simulink model "temp_sensor"  (R2025b)
settings: Solver=VariableStepAuto  StartTime=0.0  StopTime=10.0  RelTol=1e-3
undefined symbols (not defined in the file): dspblkCoreblockFVToolHelper, gcbh
libraries: arduinolib x2
settings Model: Creator=00782620  LastModifiedBy=00782620

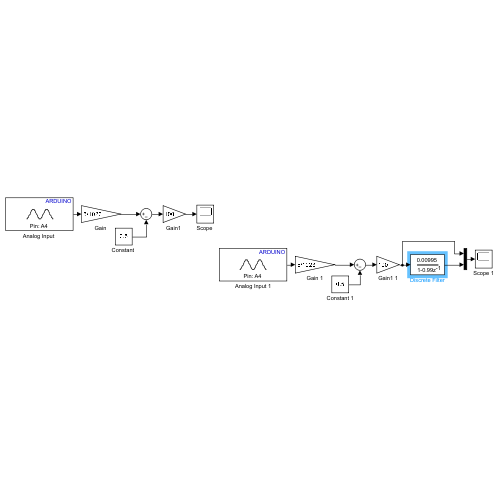
[thumbnail: Simulink's stored preview of the top-level diagram]
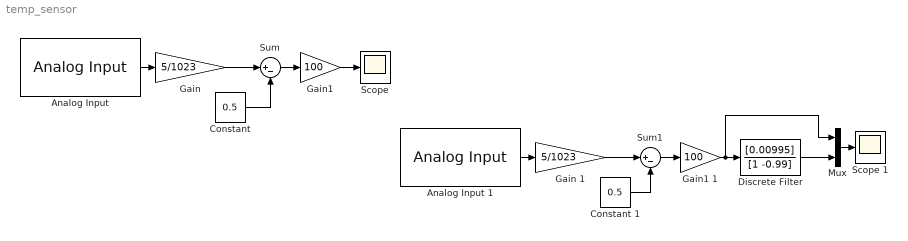
== system temp_sensor ==
  "Analog Input " : arduinolib/Analog Input  pinNumber=4  ReadResultsOnly=off  ConversionTriggerSource=Software  ExternalTriggerType=uint32( 0 )  OutputDataType=uint16  EnableConversionCompleteNotify=off  EnableOuputStatus=off  SampleTime=0.01  blockPlatform=arduino
  Analog Input 1 : arduinolib/Analog Input  pinNumber=4  ReadResultsOnly=off  ConversionTriggerSource=Software  ExternalTriggerType=uint32( 0 )  OutputDataType=uint16  EnableConversionCompleteNotify=off  EnableOuputStatus=off  SampleTime=0.01  blockPlatform=arduino
  "Constant " : Constant  Value=0.5
  Constant 1 : Constant  Value=0.5
  Discrete Filter : DiscreteFilter  LoadFcn=dspblkCoreblockFVToolHelper(gcbh,'load');  Numerator=[0.00995]  Denominator=[1 -0.99]
      settings: CopyFcn=dspblkCoreblockFVToolHelper(gcbh,'copy');  DeleteFcn=dspblkCoreblockFVToolHelper(gcbh,'close');  ModelCloseFcn=dspblkCoreblockFVToolHelper(gcbh,'close');  PreSaveFcn=dspblkCoreblockFVToolHelper(gcbh,'presave');  PostSaveFcn=dspblkCoreblockFVToolHelper(gcbh,'postsave');  CloseFcn=dspblkCoreblockFVToolHelper(gcbh,'close');
  "Gain " : Gain  Gain=5/1023
  Gain 1 : Gain  Gain=5/1023
  "Gain1 " : Gain  Gain=100
  Gain1 1 : Gain  Gain=100
  Mux : Mux  Inputs=2
  "Scope " : Scope
  Scope 1 : Scope
  Sum : Sum  Inputs=|+-
  Sum1 : Sum  Inputs=|+-
  wires:
  "Analog Input "/1 -> "Gain "/1
  "Gain "/1 -> Sum/1
  "Constant "/1 -> Sum/2
  Sum/1 -> "Gain1 "/1
  "Gain1 "/1 -> "Scope "/1
  Sum1/1 -> Gain1 1/1
  Constant 1/1 -> Sum1/2
  Gain 1/1 -> Sum1/1
  Analog Input 1/1 -> Gain 1/1
  Gain1 1/1 -> Mux/1, Discrete Filter/1
  Discrete Filter/1 -> Mux/2
  Mux/1 -> Scope 1/1
